simulink model "Controller_trorque_cbf_22Franka"  (R2022b)
settings: Solver=FixedStepDiscrete  StartTime=0.0  StopTime=inf  FixedStep=0.001  RelTol=1e-3
PreLoadFcn:
  | set_param(gcs, 'RTWSystemTargetFile', 'franka_emika_panda.tlc');
  | 
  | demos_common_configs();
  | collision_behavior = ones(1,52)*100;
values from neighbouring files (symbols this model uses):
  b_sg = fliplr(B(end, :))    [init_torque_cbf.m]
  cbf_dt = 0.001    [init_torque_cbf.m]
  cbf_Kd_rot = [120; 120; 120]*0    [init_torque_cbf.m]
  cbf_Kd_trans = [2000; 2000; 0]*0    [init_torque_cbf.m]
  cbf_stiff_decouple = 0    [init_torque_cbf.m]
  cbf_zeta_rot = [0.7; 0.7; 0.7]*0    [init_torque_cbf.m]
  cbf_zeta_trans = [0.7; 0.7; 0]*0    [init_torque_cbf.m]
  Dn = 20 * ones(7,1)    [init_torque_cbf.m]
  H_home = getTransform(Franka_robot, q_home, 'panda_link8', 'panda_link0')    [init_torque_cbf.m]
  Kn = 0 * ones(7,1)    [init_torque_cbf.m]
  plane_normal = [0.0; 0.0; 1.0]    [init_torque_cbf.m]
  q_home = q_init    [init_torque_cbf.m]
  q_init = [0 0  0  -(2/4)*pi  0  pi/2  -pi/4]'    [init_torque_cbf.m]
undefined symbols (not defined in the file or in its folder): cbf_torque_params, DiscIntNeverNeededParam, Fext_mag
libraries: franka_simulink_library x2, Robotics_lib x1, matrix_library x1
(part 5 of 7)

== matlab function Controller_trorque_cbf_22Franka/MATLAB Function ==
  data: H input; p output
function p = fcn(H)

p = H(1:3,4);

== matlab function Controller_trorque_cbf_22Franka/task space controller/MATLAB Function1 ==
  data: n_hp input; F_ext output; wrench_ext input
function F_ext = fcn(n_hp, wrench_ext)

% F_ext = (n_hp).*wrench_ext;
F_ext = wrench_ext;

end

== matlab function Controller_trorque_cbf_22Franka/MATLAB Function2 ==
  data: H_init input; H_ref output; d input; R_I_t output
function [H_ref, R_I_t] = fcn(H_init, d)

H_ref = H_init;
% H_ref(1:3,4) = d;
R_I_t = H_ref(1:3,1:3);

end
